simulink model "Assignment2"  (R2026a)
settings: Solver=VariableStepAuto  StopTime=16  MaxStep=0.001
values from neighbouring files (symbols this model uses):
  a = 0.4    [assignment2_param.m]
  b = 0.4    [assignment2_param.m]
  G = [g1 0; 0 g2]    [assignment2_param.m]
  g1 = 1    [assignment2_param.m]
  g2 = 1    [assignment2_param.m]
settings Model: Creator=saradenti  LastModifiedBy=saradenti

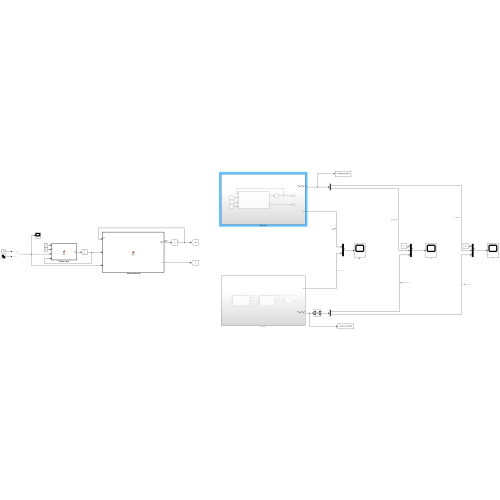
[thumbnail: Simulink's stored preview of the top-level diagram]
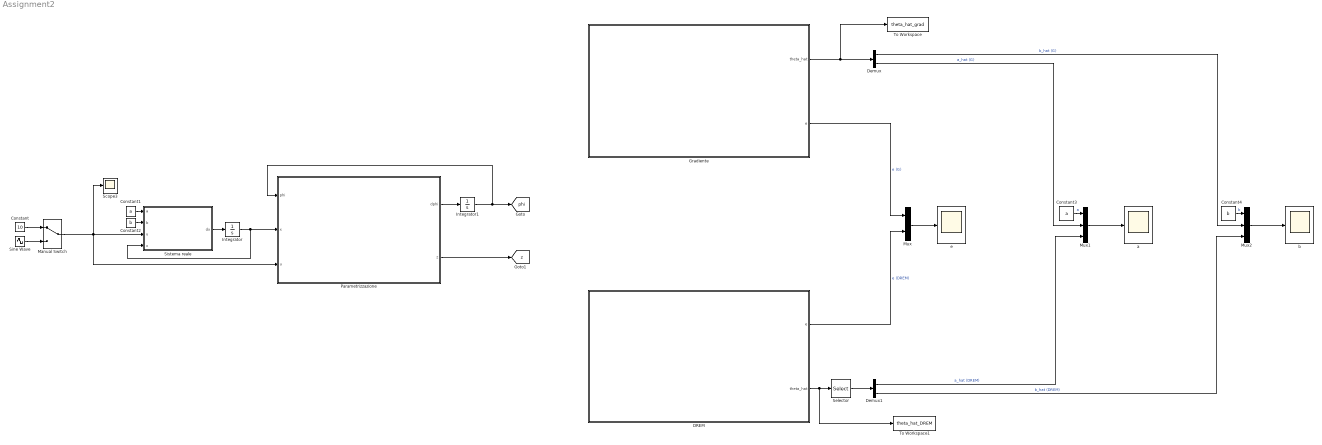
== system Assignment2 ==
  Constant : Constant  Value=10
  Constant1 : Constant  Value=a
  Constant2 : Constant  Value=b
  Constant3 : Constant  Value=a
  Constant4 : Constant  Value=b
  DREM : Subsystem
  Demux : Demux  Outputs=2
  Demux1 : Demux  Outputs=2
  Gradiente : Subsystem
  Integrator : Integrator
  Integrator1 : Integrator  InitialCondition=[0; 0]
  Manual Switch : ManualSwitch
  Mux : Mux  Inputs=2
  Mux1 : Mux  Inputs=3
  Mux2 : Mux  Inputs=3
  Parametrizzazione : MATLAB Function  TreatAsAtomicUnit=on
  Scope3 : Scope
      settings: ActiveDisplayYMinimum=-12.496292999656497  ActiveDisplayYMaximum=12.498822573728974  DataLoggingVariableName=ScopeData3
  Selector : Selector  InputPortWidth=2  IndexOptions=Index vector (dialog)  Indices=[2 1]  OutputSizes=1
  Sine Wave : Sin  Amplitude=10  Frequency=5/2  SampleTime=0
  Sistema reale : MATLAB Function  TreatAsAtomicUnit=on
  To Workspace : ToWorkspace  VariableName=theta_hat_grad  SampleTime=-1
  To Workspace1 : ToWorkspace  VariableName=theta_hat_DREM  SampleTime=-1
  a : Scope
      settings: ActiveDisplayYMinimum=6.7983980059832527E-5  ActiveDisplayYMaximum=0.22574629958777945
  b : Scope
      settings: ActiveDisplayYMinimum=0.15025691615992509  ActiveDisplayYMaximum=0.38331814158909483  DataLoggingVariableName=ScopeData2
  e : Scope
      settings: ActiveDisplayYMinimum=-2.386929776637734  ActiveDisplayYMaximum=0.28397468857736735
  tag scope: phi=global, z=global
  wires:
  Integrator/1 -> Sistema reale/4(x), Parametrizzazione/2(x)
  Sine Wave/1 -> Manual Switch/2
  Constant/1 -> Manual Switch/1
  Manual Switch/1 -> Parametrizzazione/3(u), Scope3/1, Sistema reale/3(u)
  Sistema reale/1(dx) -> Integrator/1
  Constant2/1 -> Sistema reale/2(b)
  Constant1/1 -> Sistema reale/1(a)
  Parametrizzazione/1(dphi) -> Integrator1/1
  Integrator1/1 -> Parametrizzazione/1(phi), [phi]
  Parametrizzazione/2(z) -> [z]
  Gradiente/1(theta_hat) -> Demux/1, To Workspace/1
  Gradiente/2(e) -> Mux/1  "e (G)"
  DREM/1(e) -> Mux/2  "e (DREM)"
  Mux/1 -> e/1
  Mux1/1 -> a/1
  Mux2/1 -> b/1
  Demux/1 -> Mux2/2  "b_hat (G)"
  Demux/2 -> Mux1/2  "a_hat (G)"
  Selector/1 -> Demux1/1
  Demux1/2 -> Mux2/3  "b_hat (DREM)"
  Demux1/1 -> Mux1/3  "a_hat (DREM)"
  Constant3/1 -> Mux1/1  "a"
  Constant4/1 -> Mux2/1  "b"
  DREM/2(theta_hat) -> To Workspace1/1, Selector/1

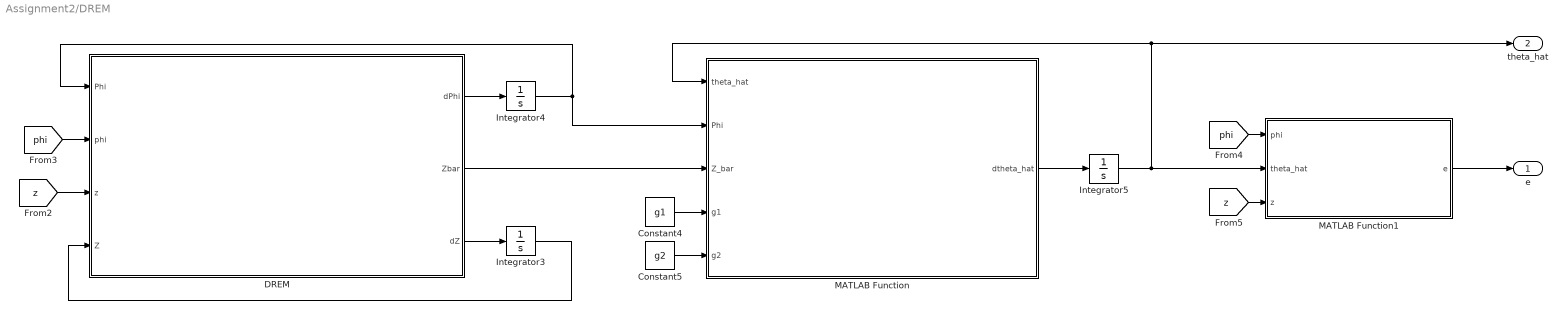
== system Assignment2/DREM ==
  Constant4 : Constant  Value=g1
  Constant5 : Constant  Value=g2
  DREM : MATLAB Function  TreatAsAtomicUnit=on
  Integrator3 : Integrator  InitialCondition=[0;0]
  Integrator4 : Integrator  InitialCondition=[0 0;0 0]
  Integrator5 : Integrator  InitialCondition=[0; 0]
  MATLAB Function : MATLAB Function  TreatAsAtomicUnit=on
  MATLAB Function1 : MATLAB Function  TreatAsAtomicUnit=on
  e : Outport
  theta_hat : Outport  Port=2
  wires:
  DREM/3(dZ) -> Integrator3/1
  [phi] -> MATLAB Function1/1(phi)
  Constant4/1 -> MATLAB Function/4(g1)
  Integrator5/1 -> theta_hat/1, MATLAB Function/1(theta_hat), MATLAB Function1/2(theta_hat)
  Integrator3/1 -> DREM/4(Z)
  [phi] -> DREM/2(phi)
  [z] -> MATLAB Function1/3(z)
  MATLAB Function1/1(e) -> e/1
  Integrator4/1 -> DREM/1(Phi), MATLAB Function/2(Phi)
  MATLAB Function/1(dtheta_hat) -> Integrator5/1
  [z] -> DREM/3(z)
  Constant5/1 -> MATLAB Function/5(g2)
  DREM/2(Zbar) -> MATLAB Function/3(Z_bar)
  DREM/1(dPhi) -> Integrator4/1

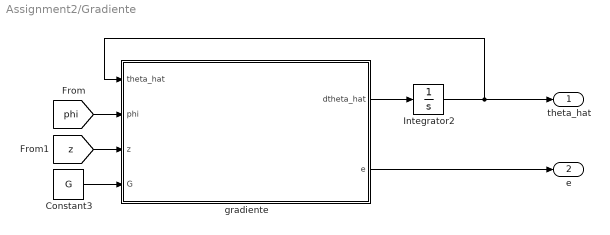
== system Assignment2/Gradiente ==
  Constant3 : Constant  Value=G
  Integrator2 : Integrator  InitialCondition=[0;0]
  gradiente : MATLAB Function  TreatAsAtomicUnit=on
  theta_hat : Outport
  e : Outport  Port=2
  wires:
  gradiente/2(e) -> e/1
  [z] -> gradiente/3(z)
  gradiente/1(dtheta_hat) -> Integrator2/1
  Constant3/1 -> gradiente/4(G)
  [phi] -> gradiente/2(phi)
  Integrator2/1 -> gradiente/1(theta_hat), theta_hat/1

== matlab function Assignment2/Parametrizzazione ==
  data: phi input; x input; u input; dphi output; z output
function [dphi,z] = fcn(phi, x, u)

    xi = phi(1);
    eta = phi(2);

    dxi = - xi + u;
    deta = - eta - x;

    dphi = [dxi; deta];
    z = x + eta;

== matlab function Assignment2/Sistema reale ==
  data: a input; b input; u input; x input; dx output
function dx = fcn(a,b, u, x)

    dx = - a * x + b * u;

== matlab function Assignment2/Gradiente/gradiente ==
  data: dtheta_hat output; theta_hat input; e output; phi input; z input; G input
function [dtheta_hat, e] = fcn(theta_hat, phi, z, G)

    e = theta_hat' * phi - z;

    dtheta_hat = - e * G * phi;

== matlab function Assignment2/DREM/DREM ==
  data: Phi input; phi input; z input; dPhi output; Zbar output; Z input; dZ output
function [dPhi,Zbar, dZ] = fcn(Phi, phi, z, Z)
    
    dZ = zeros(2,1);
    
    dZ(1) = -Z(1) + z;
    dZ(2) = - 2 * Z(2) + 2 * z;

    dPhi = [-1 0; 0 -2] * Phi + [1; 2] * phi';

    Zbar = [Phi(2,2) -Phi(1,2); -Phi(2,1) Phi(1,1)] * Z;

== matlab function Assignment2/DREM/MATLAB Function ==
  data: theta_hat input; Phi input; dtheta_hat output; Z_bar input; g1 input; g2 input
function dtheta_hat   = fcn(theta_hat, Phi, Z_bar, g1, g2)

    det_Phi = det(Phi);

    e = det_Phi * theta_hat - Z_bar;
    dtheta_hat = - det_Phi * [g1; g2] .* e;

== matlab function Assignment2/DREM/MATLAB Function1 ==
  data: phi input; theta_hat input; e output; z input
function e = fcn(phi, theta_hat, z)

    e = theta_hat' * phi - z;
